simulink model "FW_SkySurfer_HIL"  (R2026b)
settings: Solver=ode4  StopTime=inf  FixedStep=Thil  EnableMultiTasking=on
PreLoadFcn:
  | % Load this folder's HIL settings and MAVLink Bus types (not another project's).
  | run(fullfile(fileparts(get_param(bdroot,'FileName')),'PX4_HIL_preload.m'));
InitFcn:
  | % Record the model first: loading libraries can change the current diagram.
  | assignin('base','lastRunModel',bdroot);
  | % Rebuild HIL settings/Bus types (also after clear all), then aircraft data.
  | hilModelFolder = fileparts(get_param(lastRunModel,'FileName'));
  | run(fullfile(hilModelFolder,'PX4_HIL_preload.m'));
  | run(fullfile(hilModelFolder,'FW_SkySurfer_InitialFunction.m'));
  | clear hilModelFolder
values from neighbouring files (symbols this model uses):
  Aeroelasticity_AIL = [   5   15]    [FW_SkySurfer_InitialFunction.m]
  Aeroelasticity_ELE = [   5   15]    [FW_SkySurfer_InitialFunction.m]
  Aeroelasticity_Gain_AIL = [ 0.8  0.5]    [FW_SkySurfer_InitialFunction.m]
  Aeroelasticity_Gain_ELE = [ 0.9  0.6]    [FW_SkySurfer_InitialFunction.m]
  Aeroelasticity_Gain_RUD = [ 0.9  0.6]    [FW_SkySurfer_InitialFunction.m]
  Aeroelasticity_RUD = [   5   15]    [FW_SkySurfer_InitialFunction.m]
  alpha_avl = [-10 -5 0 5 10 15]    [import_aerostates_avl.m]
  AoA = [-10 -5 0 5 10 15]    [import_aerostates_vsp.m]
  AoS = [-10 0 10]    [import_aerostates_vsp.m]
  b = 1.41    [FW_SkySurfer_InitialFunction.m]
  beta_avl = [-10 -5 0 5 10]    [import_aerostates_avl.m]
  C_wgrp = struct()    [import_aerostates_vsp.m]
  cbar = 0.20    (= 0.2)    [FW_SkySurfer_InitialFunction.m]
  CD_fix_AVL = 0.075    [FW_SkySurfer_InitialFunction.m]
  CD_fix_VSP = 0.065    [FW_SkySurfer_InitialFunction.m]
  CDd01 = zeros(length(mach_avl), length(alpha_avl), length(beta_avl))    [import_aerostates_avl.m]
  CDd02 = zeros(length(mach_avl), length(alpha_avl), length(beta_avl))    [import_aerostates_avl.m]
  CDd03 = zeros(length(mach_avl), length(alpha_avl), length(beta_avl))    [import_aerostates_avl.m]
  CDd04 = zeros(length(mach_avl), length(alpha_avl), length(beta_avl))    [import_aerostates_avl.m]
  CDp = zeros(length(mach_avl), length(alpha_avl), length(beta_avl))    [import_aerostates_avl.m]
  CDq = zeros(length(mach_avl), length(alpha_avl), length(beta_avl))    [import_aerostates_avl.m]
  CDr = zeros(length(mach_avl), length(alpha_avl), length(beta_avl))    [import_aerostates_avl.m]
  CDtot = zeros(length(mach_avl), length(alpha_avl), length(beta_avl))    [import_aerostates_avl.m]
  CG_m = [0.330, 0, 0]    [FW_SkySurfer_InitialFunction.m]
  CLd01 = zeros(length(mach_avl), length(alpha_avl), length(beta_avl))    [import_aerostates_avl.m]
  Cld01 = zeros(length(mach_avl), length(alpha_avl), length(beta_avl))    [import_aerostates_avl.m]
  CLd02 = zeros(length(mach_avl), length(alpha_avl), length(beta_avl))    [import_aerostates_avl.m]
  Cld02 = zeros(length(mach_avl), length(alpha_avl), length(beta_avl))    [import_aerostates_avl.m]
  CLd03 = zeros(length(mach_avl), length(alpha_avl), length(beta_avl))    [import_aerostates_avl.m]
  Cld03 = zeros(length(mach_avl), length(alpha_avl), length(beta_avl))    [import_aerostates_avl.m]
  CLd04 = zeros(length(mach_avl), length(alpha_avl), length(beta_avl))    [import_aerostates_avl.m]
  Cld04 = zeros(length(mach_avl), length(alpha_avl), length(beta_avl))    [import_aerostates_avl.m]
  CLp = zeros(length(mach_avl), length(alpha_avl), length(beta_avl))    [import_aerostates_avl.m]
  Clp = zeros(length(mach_avl), length(alpha_avl), length(beta_avl))    [import_aerostates_avl.m]
  CLq = zeros(length(mach_avl), length(alpha_avl), length(beta_avl))    [import_aerostates_avl.m]
  Clq = zeros(length(mach_avl), length(alpha_avl), length(beta_avl))    [import_aerostates_avl.m]
  CLr = zeros(length(mach_avl), length(alpha_avl), length(beta_avl))    [import_aerostates_avl.m]
  Clr = zeros(length(mach_avl), length(alpha_avl), length(beta_avl))    [import_aerostates_avl.m]
  CLtot = zeros(length(mach_avl), length(alpha_avl), length(beta_avl))    [import_aerostates_avl.m]
  Cltot = zeros(length(mach_avl), length(alpha_avl), length(beta_avl))    [import_aerostates_avl.m]
  Cmd01 = zeros(length(mach_avl), length(alpha_avl), length(beta_avl))    [import_aerostates_avl.m]
  Cmd02 = zeros(length(mach_avl), length(alpha_avl), length(beta_avl))    [import_aerostates_avl.m]
  Cmd03 = zeros(length(mach_avl), length(alpha_avl), length(beta_avl))    [import_aerostates_avl.m]
  Cmd04 = zeros(length(mach_avl), length(alpha_avl), length(beta_avl))    [import_aerostates_avl.m]
  Cmp = zeros(length(mach_avl), length(alpha_avl), length(beta_avl))    [import_aerostates_avl.m]
  Cmq = zeros(length(mach_avl), length(alpha_avl), length(beta_avl))    [import_aerostates_avl.m]
  Cmr = zeros(length(mach_avl), length(alpha_avl), length(beta_avl))    [import_aerostates_avl.m]
  Cmtot = zeros(length(mach_avl), length(alpha_avl), length(beta_avl))    [import_aerostates_avl.m]
  Cnd01 = zeros(length(mach_avl), length(alpha_avl), length(beta_avl))    [import_aerostates_avl.m]
  Cnd02 = zeros(length(mach_avl), length(alpha_avl), length(beta_avl))    [import_aerostates_avl.m]
  Cnd03 = zeros(length(mach_avl), length(alpha_avl), length(beta_avl))    [import_aerostates_avl.m]
  Cnd04 = zeros(length(mach_avl), length(alpha_avl), length(beta_avl))    [import_aerostates_avl.m]
  Cnp = zeros(length(mach_avl), length(alpha_avl), length(beta_avl))    [import_aerostates_avl.m]
  Cnq = zeros(length(mach_avl), length(alpha_avl), length(beta_avl))    [import_aerostates_avl.m]
  Cnr = zeros(length(mach_avl), length(alpha_avl), length(beta_avl))    [import_aerostates_avl.m]
  Cntot = zeros(length(mach_avl), length(alpha_avl), length(beta_avl))    [import_aerostates_avl.m]
  CYd01 = zeros(length(mach_avl), length(alpha_avl), length(beta_avl))    [import_aerostates_avl.m]
  CYd02 = zeros(length(mach_avl), length(alpha_avl), length(beta_avl))    [import_aerostates_avl.m]
  CYd03 = zeros(length(mach_avl), length(alpha_avl), length(beta_avl))    [import_aerostates_avl.m]
  CYd04 = zeros(length(mach_avl), length(alpha_avl), length(beta_avl))    [import_aerostates_avl.m]
  CYp = zeros(length(mach_avl), length(alpha_avl), length(beta_avl))    [import_aerostates_avl.m]
  CYq = zeros(length(mach_avl), length(alpha_avl), length(beta_avl))    [import_aerostates_avl.m]
  CYr = zeros(length(mach_avl), length(alpha_avl), length(beta_avl))    [import_aerostates_avl.m]
  CYtot = zeros(length(mach_avl), length(alpha_avl), length(beta_avl))    [import_aerostates_avl.m]
  del_z = 0    [FW_SkySurfer_InitialFunction.m]
  g = 9.80665    [FW_SkySurfer_InitialFunction.m]
  H0 = 1000 * convlength(1, 'ft', 'm')    [FW_SkySurfer_InitialFunction.m]
  Inertia0 = [  Ixx -Ixy -Ixz  ;                              -Ixy  Iyy -Iyz  ;                              -Ixz -Iyz  Izz ]    [FW_SkySurfer_InitialFunction.m]
  Lat0 = 22.910275834988674    (= 22.910275835)    [FW_SkySurfer_InitialFunction.m]
  Lon0 = 120.31096929726908    (= 120.310969297)    [FW_SkySurfer_InitialFunction.m]
  Mach = [0.05 0.10]    [import_aerostates_vsp.m]
  mach_avl = [0.05 0.10]    [import_aerostates_avl.m]
  Mass0 = 1.3    [FW_SkySurfer_InitialFunction.m]
  Phi0 = 0    [FW_SkySurfer_InitialFunction.m]
  Psi0 = 0    [FW_SkySurfer_InitialFunction.m]
  Psi_w = 0    [FW_SkySurfer_InitialFunction.m]
  Theta0 = 0.8633    [FW_SkySurfer_InitialFunction.m]
  Thil = 1/250    (= 0.004)    [FW_SkySurfer_InitialFunction.m]
  U0 = 40.0309 * convvel(1, 'kts', 'm/s')    [FW_SkySurfer_InitialFunction.m]
  useAVL_VSP = 0    [FW_SkySurfer_InitialFunction.m]
  V0 = 0    [FW_SkySurfer_InitialFunction.m]
  Vel_w = 0    [FW_SkySurfer_InitialFunction.m]
  W0 = 0.6032 * convvel(1, 'kts', 'm/s')    [FW_SkySurfer_InitialFunction.m]
  XREF_m = [0.330, 0, 0]    [FW_SkySurfer_InitialFunction.m]
undefined symbols (not defined in the file or in its folder): F, Light, m, MIL, Newton, Raphson, s, Ts, uavData
libraries: simulink_extras x28, aerolibasang x5, shared6dofsys x4, aerolibwind2 x4, sharedtransform x3, sharedutil x2, shared6dof x2, simulink x1, aerolibatmos2 x1, aerolibconvert2 x1
(part 2 of 3)

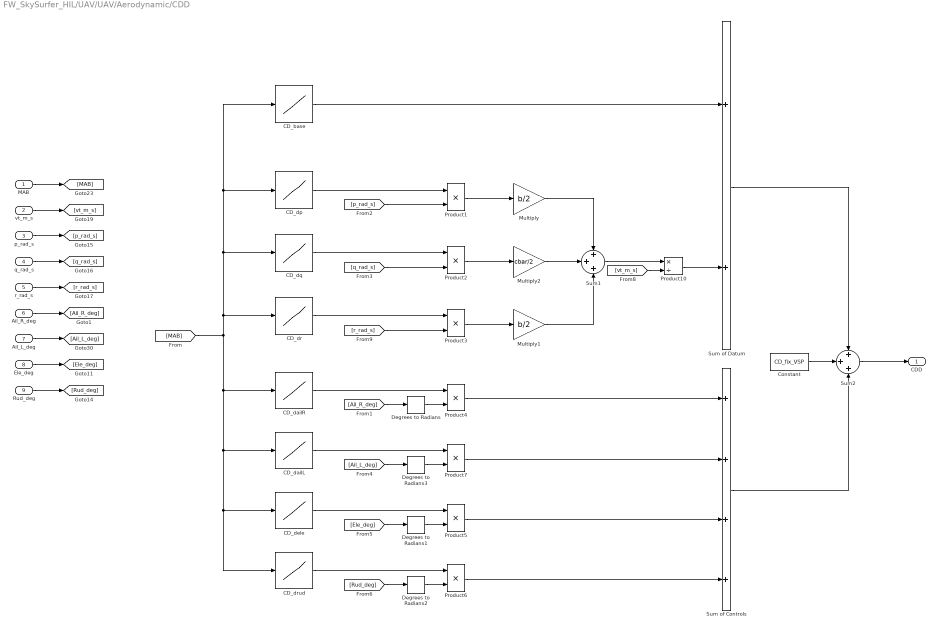
== system FW_SkySurfer_HIL/UAV/UAV/Aerodynamic/CDD ==
  MAB : Inport
  vt_m_s : Inport  Port=2
  p_rad_s : Inport  Port=3
  q_rad_s : Inport  Port=4
  r_rad_s : Inport  Port=5
  Ail_R_deg : Inport  Port=6
  Ail_L_deg : Inport  Port=7
  Ele_deg : Inport  Port=8
  Rud_deg : Inport  Port=9
  CD_base : Lookup_n-D  NumberOfTableDimensions=3  BreakpointsForDimension1=Mach  BreakpointsForDimension2=AoA  BreakpointsForDimension3=AoS  UseOneInputPortForAllInputData=on  Table=C_wgrp.CD_wgrp{1}  InternalRulePriority=Speed  RndMeth=Simplest
  CD_dailL : Lookup_n-D  NumberOfTableDimensions=3  BreakpointsForDimension1=Mach  BreakpointsForDimension2=AoA  BreakpointsForDimension3=AoS  UseOneInputPortForAllInputData=on  Table=C_wgrp.CD_wgrp{10}  InternalRulePriority=Speed  RndMeth=Simplest
  CD_dailR : Lookup_n-D  NumberOfTableDimensions=3  BreakpointsForDimension1=Mach  BreakpointsForDimension2=AoA  BreakpointsForDimension3=AoS  UseOneInputPortForAllInputData=on  Table=C_wgrp.CD_wgrp{9}  InternalRulePriority=Speed  RndMeth=Simplest
  CD_dele : Lookup_n-D  NumberOfTableDimensions=3  BreakpointsForDimension1=Mach  BreakpointsForDimension2=AoA  BreakpointsForDimension3=AoS  UseOneInputPortForAllInputData=on  Table=C_wgrp.CD_wgrp{11}  InternalRulePriority=Speed  RndMeth=Simplest
  CD_dp : Lookup_n-D  NumberOfTableDimensions=3  BreakpointsForDimension1=Mach  BreakpointsForDimension2=AoA  BreakpointsForDimension3=AoS  UseOneInputPortForAllInputData=on  Table=C_wgrp.CD_wgrp{4}  InternalRulePriority=Speed  RndMeth=Simplest
  CD_dq : Lookup_n-D  NumberOfTableDimensions=3  BreakpointsForDimension1=Mach  BreakpointsForDimension2=AoA  BreakpointsForDimension3=AoS  UseOneInputPortForAllInputData=on  Table=C_wgrp.CD_wgrp{5}  InternalRulePriority=Speed  RndMeth=Simplest
  CD_dr : Lookup_n-D  NumberOfTableDimensions=3  BreakpointsForDimension1=Mach  BreakpointsForDimension2=AoA  BreakpointsForDimension3=AoS  UseOneInputPortForAllInputData=on  Table=C_wgrp.CD_wgrp{6}  InternalRulePriority=Speed  RndMeth=Simplest
  CD_drud : Lookup_n-D  NumberOfTableDimensions=3  BreakpointsForDimension1=Mach  BreakpointsForDimension2=AoA  BreakpointsForDimension3=AoS  UseOneInputPortForAllInputData=on  Table=C_wgrp.CD_wgrp{12}  InternalRulePriority=Speed  RndMeth=Simplest
  Constant : Constant  Value=CD_fix_VSP
  Degrees to Radians{,1..3} (4 alike) : simulink_extras/Transformations/Degrees to Radians
  Multiply : Gain  Gain=b/2
  Multiply1 : Gain  Gain=b/2
  Multiply2 : Gain  Gain=cbar/2
  Product{1..7} (7 alike) : Product
  Product10 : Product  Inputs=*/  InputSameDT=on  SaturateOnIntegerOverflow=on  OutDataTypeStr=Inherit: Same as first input
  Sum of Controls : Sum  Inputs=++++
  Sum of Datum : Sum
  Sum1 : Sum  Inputs=+++  InputSameDT=on  SaturateOnIntegerOverflow=on  OutDataTypeStr=Inherit: Same as first input
  Sum2 : Sum  Inputs=+++  InputSameDT=on  SaturateOnIntegerOverflow=on  OutDataTypeStr=Inherit: Same as first input
  CDD : Outport
  wires:
  vt_m_s/1 -> [vt_m_s]
  MAB/1 -> [MAB]
  p_rad_s/1 -> [p_rad_s]
  q_rad_s/1 -> [q_rad_s]
  r_rad_s/1 -> [r_rad_s]
  Ail_R_deg/1 -> [Ail_R_deg]
  Ail_L_deg/1 -> [Ail_L_deg]
  Ele_deg/1 -> [Ele_deg]
  Rud_deg/1 -> [Rud_deg]
  Sum2/1 -> CDD/1
  CD_dailR/1 -> Product4/1
  Multiply/1 -> Sum1/1
  Sum of Controls/1 -> Sum2/3
  Degrees to Radians1/1 -> Product5/2
  Degrees to Radians3/1 -> Product7/2
  CD_drud/1 -> Product6/1
  CD_dr/1 -> Product3/1
  Product7/1 -> Sum of Controls/2
  Product5/1 -> Sum of Controls/3
  CD_dq/1 -> Product2/1
  Sum of Datum/1 -> Sum2/1
  Product3/1 -> Multiply1/1
  CD_dp/1 -> Product1/1
  Multiply2/1 -> Sum1/2
  Degrees to Radians2/1 -> Product6/2
  CD_base/1 -> Sum of Datum/1
  Multiply1/1 -> Sum1/3
  Product6/1 -> Sum of Controls/4
  Product2/1 -> Multiply2/1
  [p_rad_s] -> Product1/2
  Product1/1 -> Multiply/1
  [Ail_L_deg] -> Degrees to Radians3/1
  [Ele_deg] -> Degrees to Radians1/1
  Product10/1 -> Sum of Datum/2
  Degrees to Radians/1 -> Product4/2
  CD_dailL/1 -> Product7/1
  Product4/1 -> Sum of Controls/1
  [Rud_deg] -> Degrees to Radians2/1
  [r_rad_s] -> Product3/2
  [vt_m_s] -> Product10/2
  [MAB] -> CD_dq/1, CD_base/1, CD_dp/1, CD_dr/1, CD_dele/1, CD_drud/1, CD_dailL/1, CD_dailR/1
  CD_dele/1 -> Product5/1
  [q_rad_s] -> Product2/2
  [Ail_R_deg] -> Degrees to Radians/1
  Constant/1 -> Sum2/2
  Sum1/1 -> Product10/1

== system FW_SkySurfer_HIL/UAV/UAV/Aerodynamic/CL ==
  MAB : Inport
  vt_m_s : Inport  Port=2
  p_rad_s : Inport  Port=3
  q_rad_s : Inport  Port=4
  r_rad_s : Inport  Port=5
  Ail_R_deg : Inport  Port=6
  Ail_L_deg : Inport  Port=7
  Ele_deg : Inport  Port=8
  Rud_deg : Inport  Port=9
  CLd01 : Lookup_n-D  NumberOfTableDimensions=3  BreakpointsForDimension1=mach_avl  BreakpointsForDimension2=alpha_avl  BreakpointsForDimension3=beta_avl  UseOneInputPortForAllInputData=on  Table=CLd01  InternalRulePriority=Speed  RndMeth=Simplest
  CLd02 : Lookup_n-D  NumberOfTableDimensions=3  BreakpointsForDimension1=mach_avl  BreakpointsForDimension2=alpha_avl  BreakpointsForDimension3=beta_avl  UseOneInputPortForAllInputData=on  Table=CLd02  InternalRulePriority=Speed  RndMeth=Simplest
  CLd03 : Lookup_n-D  NumberOfTableDimensions=3  BreakpointsForDimension1=mach_avl  BreakpointsForDimension2=alpha_avl  BreakpointsForDimension3=beta_avl  UseOneInputPortForAllInputData=on  Table=CLd03  InternalRulePriority=Speed  RndMeth=Simplest
  CLd04 : Lookup_n-D  NumberOfTableDimensions=3  BreakpointsForDimension1=mach_avl  BreakpointsForDimension2=alpha_avl  BreakpointsForDimension3=beta_avl  UseOneInputPortForAllInputData=on  Table=CLd04  InternalRulePriority=Speed  RndMeth=Simplest
  CLp : Lookup_n-D  NumberOfTableDimensions=3  BreakpointsForDimension1=mach_avl  BreakpointsForDimension2=alpha_avl  BreakpointsForDimension3=beta_avl  UseOneInputPortForAllInputData=on  Table=CLp  InternalRulePriority=Speed  RndMeth=Simplest
  CLq : Lookup_n-D  NumberOfTableDimensions=3  BreakpointsForDimension1=mach_avl  BreakpointsForDimension2=alpha_avl  BreakpointsForDimension3=beta_avl  UseOneInputPortForAllInputData=on  Table=CLq  InternalRulePriority=Speed  RndMeth=Simplest
  CLr : Lookup_n-D  NumberOfTableDimensions=3  BreakpointsForDimension1=mach_avl  BreakpointsForDimension2=alpha_avl  BreakpointsForDimension3=beta_avl  UseOneInputPortForAllInputData=on  Table=CLr  InternalRulePriority=Speed  RndMeth=Simplest
  CLtot : Lookup_n-D  NumberOfTableDimensions=3  BreakpointsForDimension1=mach_avl  BreakpointsForDimension2=alpha_avl  BreakpointsForDimension3=beta_avl  UseOneInputPortForAllInputData=on  Table=CLtot  InternalRulePriority=Speed  RndMeth=Simplest
  Multiply : Gain  Gain=b/2
  Multiply1 : Gain  Gain=b/2
  Multiply2 : Gain  Gain=cbar/2
  Product{1..7} (7 alike) : Product
  Product10 : Product  Inputs=*/  InputSameDT=on  SaturateOnIntegerOverflow=on  OutDataTypeStr=Inherit: Same as first input
  Sum of Controls : Sum  Inputs=++++
  Sum of Datum : Sum
  Sum1 : Sum  Inputs=+++  InputSameDT=on  SaturateOnIntegerOverflow=on  OutDataTypeStr=Inherit: Same as first input
  Sum4 : Sum  InputSameDT=on  SaturateOnIntegerOverflow=on  OutDataTypeStr=Inherit: Same as first input
  CL : Outport
  wires:
  q_rad_s/1 -> [q_rad_s]
  vt_m_s/1 -> [vt_m_s]
  p_rad_s/1 -> [p_rad_s]
  Ail_L_deg/1 -> [Ail_L_deg]
  Ail_R_deg/1 -> [Ail_R_deg]
  MAB/1 -> [MAB]
  r_rad_s/1 -> [r_rad_s]
  Rud_deg/1 -> [Rud_deg]
  Ele_deg/1 -> [Ele_deg]
  [MAB] -> CLr/1, CLq/1, CLp/1, CLtot/1, CLd01/1, CLd02/1, CLd04/1, CLd03/1
  CLd02/1 -> Product7/1
  CLd04/1 -> Product6/1
  Product7/1 -> Sum of Controls/2
  Sum4/1 -> CL/1
  CLd01/1 -> Product4/1
  [r_rad_s] -> Product3/2
  Multiply/1 -> Sum1/1
  Product5/1 -> Sum of Controls/3
  Multiply1/1 -> Sum1/3
  [vt_m_s] -> Product10/2
  Sum of Controls/1 -> Sum4/2
  CLd03/1 -> Product5/1
  Product2/1 -> Multiply2/1
  CLtot/1 -> Sum of Datum/1
  CLq/1 -> Product2/1
  [p_rad_s] -> Product1/2
  Product3/1 -> Multiply1/1
  Product6/1 -> Sum of Controls/4
  Sum of Datum/1 -> Sum4/1
  CLp/1 -> Product1/1
  [q_rad_s] -> Product2/2
  Product1/1 -> Multiply/1
  Multiply2/1 -> Sum1/2
  Product10/1 -> Sum of Datum/2
  CLr/1 -> Product3/1
  Product4/1 -> Sum of Controls/1
  Sum1/1 -> Product10/1
  [Ail_L_deg] -> Product7/2
  [Rud_deg] -> Product6/2
  [Ele_deg] -> Product5/2
  [Ail_R_deg] -> Product4/2

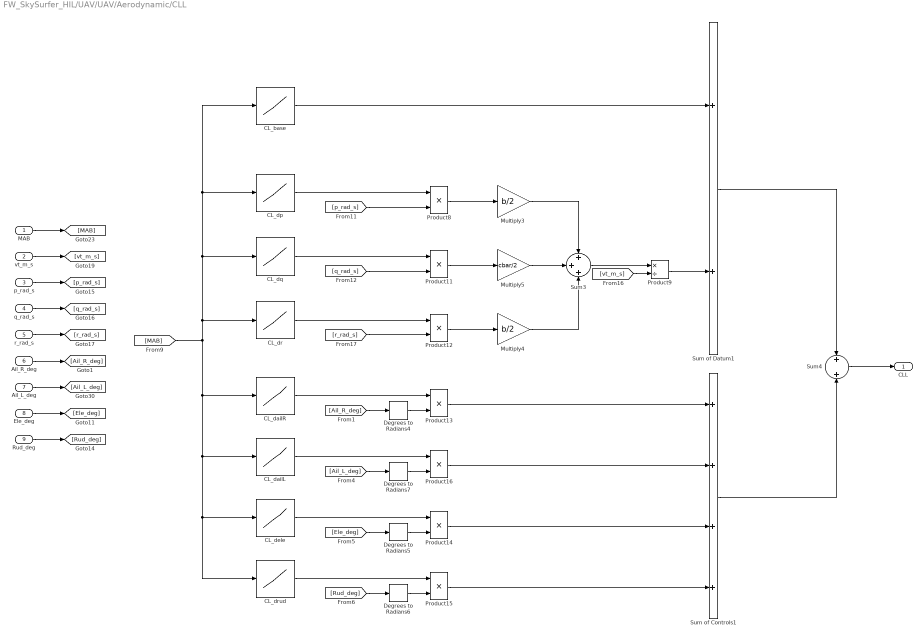
== system FW_SkySurfer_HIL/UAV/UAV/Aerodynamic/CLL ==
  MAB : Inport
  vt_m_s : Inport  Port=2
  p_rad_s : Inport  Port=3
  q_rad_s : Inport  Port=4
  r_rad_s : Inport  Port=5
  Ail_R_deg : Inport  Port=6
  Ail_L_deg : Inport  Port=7
  Ele_deg : Inport  Port=8
  Rud_deg : Inport  Port=9
  CL_base : Lookup_n-D  NumberOfTableDimensions=3  BreakpointsForDimension1=Mach  BreakpointsForDimension2=AoA  BreakpointsForDimension3=AoS  UseOneInputPortForAllInputData=on  Table=C_wgrp.CL_wgrp{1}  InternalRulePriority=Speed  RndMeth=Simplest
  CL_dailL : Lookup_n-D  NumberOfTableDimensions=3  BreakpointsForDimension1=Mach  BreakpointsForDimension2=AoA  BreakpointsForDimension3=AoS  UseOneInputPortForAllInputData=on  Table=C_wgrp.CL_wgrp{10}  InternalRulePriority=Speed  RndMeth=Simplest
  CL_dailR : Lookup_n-D  NumberOfTableDimensions=3  BreakpointsForDimension1=Mach  BreakpointsForDimension2=AoA  BreakpointsForDimension3=AoS  UseOneInputPortForAllInputData=on  Table=C_wgrp.CL_wgrp{9}  InternalRulePriority=Speed  RndMeth=Simplest
  CL_dele : Lookup_n-D  NumberOfTableDimensions=3  BreakpointsForDimension1=Mach  BreakpointsForDimension2=AoA  BreakpointsForDimension3=AoS  UseOneInputPortForAllInputData=on  Table=C_wgrp.CL_wgrp{11}  InternalRulePriority=Speed  RndMeth=Simplest
  CL_dp : Lookup_n-D  NumberOfTableDimensions=3  BreakpointsForDimension1=Mach  BreakpointsForDimension2=AoA  BreakpointsForDimension3=AoS  UseOneInputPortForAllInputData=on  Table=C_wgrp.CL_wgrp{4}  InternalRulePriority=Speed  RndMeth=Simplest
  CL_dq : Lookup_n-D  NumberOfTableDimensions=3  BreakpointsForDimension1=Mach  BreakpointsForDimension2=AoA  BreakpointsForDimension3=AoS  UseOneInputPortForAllInputData=on  Table=C_wgrp.CL_wgrp{5}  InternalRulePriority=Speed  RndMeth=Simplest
  CL_dr : Lookup_n-D  NumberOfTableDimensions=3  BreakpointsForDimension1=Mach  BreakpointsForDimension2=AoA  BreakpointsForDimension3=AoS  UseOneInputPortForAllInputData=on  Table=C_wgrp.CL_wgrp{6}  InternalRulePriority=Speed  RndMeth=Simplest
  CL_drud : Lookup_n-D  NumberOfTableDimensions=3  BreakpointsForDimension1=Mach  BreakpointsForDimension2=AoA  BreakpointsForDimension3=AoS  UseOneInputPortForAllInputData=on  Table=C_wgrp.CL_wgrp{12}  InternalRulePriority=Speed  RndMeth=Simplest
  Degrees to Radians{4..7} (4 alike) : simulink_extras/Transformations/Degrees to Radians
  Multiply3 : Gain  Gain=b/2
  Multiply4 : Gain  Gain=b/2
  Multiply5 : Gain  Gain=cbar/2
  Product{8,11..16} (7 alike) : Product
  Product9 : Product  Inputs=*/  InputSameDT=on  SaturateOnIntegerOverflow=on  OutDataTypeStr=Inherit: Same as first input
  Sum of Controls1 : Sum  Inputs=++++
  Sum of Datum1 : Sum
  Sum3 : Sum  Inputs=+++  InputSameDT=on  SaturateOnIntegerOverflow=on  OutDataTypeStr=Inherit: Same as first input
  Sum4 : Sum  InputSameDT=on  SaturateOnIntegerOverflow=on  OutDataTypeStr=Inherit: Same as first input
  CLL : Outport
  wires:
  Ele_deg/1 -> [Ele_deg]
  q_rad_s/1 -> [q_rad_s]
  p_rad_s/1 -> [p_rad_s]
  r_rad_s/1 -> [r_rad_s]
  MAB/1 -> [MAB]
  vt_m_s/1 -> [vt_m_s]
  Rud_deg/1 -> [Rud_deg]
  Ail_L_deg/1 -> [Ail_L_deg]
  Ail_R_deg/1 -> [Ail_R_deg]
  [r_rad_s] -> Product12/2
  CL_dq/1 -> Product11/1
  Product16/1 -> Sum of Controls1/2
  Sum of Controls1/1 -> Sum4/2
  Degrees to Radians6/1 -> Product15/2
  Product15/1 -> Sum of Controls1/4
  CL_dp/1 -> Product8/1
  Multiply4/1 -> Sum3/3
  Sum of Datum1/1 -> Sum4/1
  CL_dele/1 -> Product14/1
  [Rud_deg] -> Degrees to Radians6/1
  [MAB] -> CL_dr/1, CL_dq/1, CL_dp/1, CL_base/1, CL_dailR/1, CL_dailL/1, CL_drud/1, CL_dele/1
  Product14/1 -> Sum of Controls1/3
  CL_drud/1 -> Product15/1
  CL_base/1 -> Sum of Datum1/1
  [Ele_deg] -> Degrees to Radians5/1
  Product11/1 -> Multiply5/1
  Multiply5/1 -> Sum3/2
  Product9/1 -> Sum of Datum1/2
  [vt_m_s] -> Product9/2
  Degrees to Radians4/1 -> Product13/2
  CL_dailR/1 -> Product13/1
  CL_dr/1 -> Product12/1
  [Ail_R_deg] -> Degrees to Radians4/1
  Product12/1 -> Multiply4/1
  [q_rad_s] -> Product11/2
  Sum3/1 -> Product9/1
  Product8/1 -> Multiply3/1
  Degrees to Radians7/1 -> Product16/2
  Sum4/1 -> CLL/1
  Degrees to Radians5/1 -> Product14/2
  [p_rad_s] -> Product8/2
  [Ail_L_deg] -> Degrees to Radians7/1
  Multiply3/1 -> Sum3/1
  CL_dailL/1 -> Product16/1
  Product13/1 -> Sum of Controls1/1

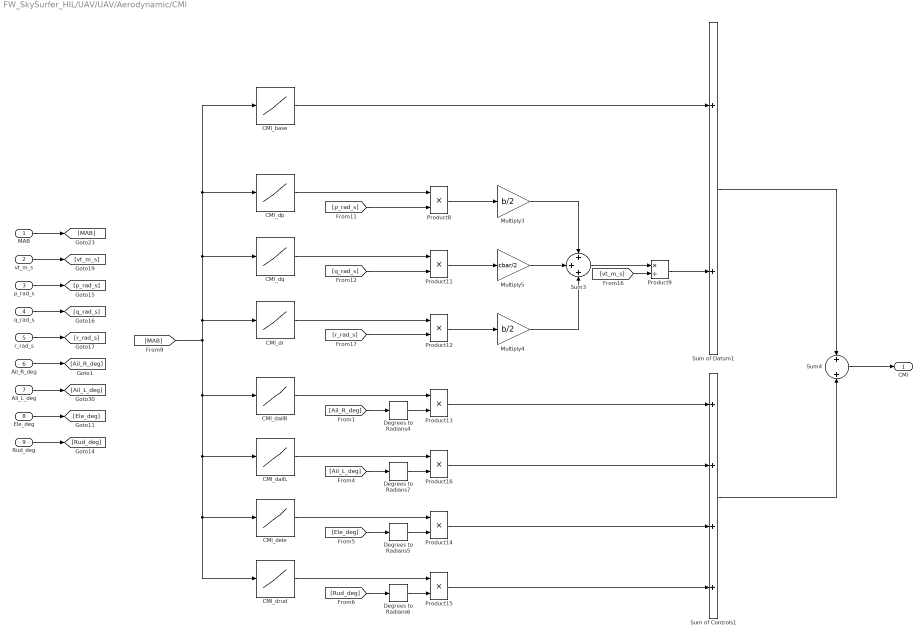
== system FW_SkySurfer_HIL/UAV/UAV/Aerodynamic/CMl ==
  MAB : Inport
  vt_m_s : Inport  Port=2
  p_rad_s : Inport  Port=3
  q_rad_s : Inport  Port=4
  r_rad_s : Inport  Port=5
  Ail_R_deg : Inport  Port=6
  Ail_L_deg : Inport  Port=7
  Ele_deg : Inport  Port=8
  Rud_deg : Inport  Port=9
  CMl_base : Lookup_n-D  NumberOfTableDimensions=3  BreakpointsForDimension1=Mach  BreakpointsForDimension2=AoA  BreakpointsForDimension3=AoS  UseOneInputPortForAllInputData=on  Table=C_wgrp.CMl_wgrp{1}  InternalRulePriority=Speed  RndMeth=Simplest
  CMl_dailL : Lookup_n-D  NumberOfTableDimensions=3  BreakpointsForDimension1=Mach  BreakpointsForDimension2=AoA  BreakpointsForDimension3=AoS  UseOneInputPortForAllInputData=on  Table=C_wgrp.CMl_wgrp{10}  InternalRulePriority=Speed  RndMeth=Simplest
  CMl_dailR : Lookup_n-D  NumberOfTableDimensions=3  BreakpointsForDimension1=Mach  BreakpointsForDimension2=AoA  BreakpointsForDimension3=AoS  UseOneInputPortForAllInputData=on  Table=C_wgrp.CMl_wgrp{9}  InternalRulePriority=Speed  RndMeth=Simplest
  CMl_dele : Lookup_n-D  NumberOfTableDimensions=3  BreakpointsForDimension1=Mach  BreakpointsForDimension2=AoA  BreakpointsForDimension3=AoS  UseOneInputPortForAllInputData=on  Table=C_wgrp.CMl_wgrp{11}  InternalRulePriority=Speed  RndMeth=Simplest
  CMl_dp : Lookup_n-D  NumberOfTableDimensions=3  BreakpointsForDimension1=Mach  BreakpointsForDimension2=AoA  BreakpointsForDimension3=AoS  UseOneInputPortForAllInputData=on  Table=C_wgrp.CMl_wgrp{4}  InternalRulePriority=Speed  RndMeth=Simplest
  CMl_dq : Lookup_n-D  NumberOfTableDimensions=3  BreakpointsForDimension1=Mach  BreakpointsForDimension2=AoA  BreakpointsForDimension3=AoS  UseOneInputPortForAllInputData=on  Table=C_wgrp.CMl_wgrp{5}  InternalRulePriority=Speed  RndMeth=Simplest
  CMl_dr : Lookup_n-D  NumberOfTableDimensions=3  BreakpointsForDimension1=Mach  BreakpointsForDimension2=AoA  BreakpointsForDimension3=AoS  UseOneInputPortForAllInputData=on  Table=C_wgrp.CMl_wgrp{6}  InternalRulePriority=Speed  RndMeth=Simplest
  CMl_drud : Lookup_n-D  NumberOfTableDimensions=3  BreakpointsForDimension1=Mach  BreakpointsForDimension2=AoA  BreakpointsForDimension3=AoS  UseOneInputPortForAllInputData=on  Table=C_wgrp.CMl_wgrp{12}  InternalRulePriority=Speed  RndMeth=Simplest
  Degrees to Radians{4..7} (4 alike) : simulink_extras/Transformations/Degrees to Radians
  Multiply3 : Gain  Gain=b/2
  Multiply4 : Gain  Gain=b/2
  Multiply5 : Gain  Gain=cbar/2
  Product{8,11..16} (7 alike) : Product
  Product9 : Product  Inputs=*/  InputSameDT=on  SaturateOnIntegerOverflow=on  OutDataTypeStr=Inherit: Same as first input
  Sum of Controls1 : Sum  Inputs=++++
  Sum of Datum1 : Sum
  Sum3 : Sum  Inputs=+++  InputSameDT=on  SaturateOnIntegerOverflow=on  OutDataTypeStr=Inherit: Same as first input
  Sum4 : Sum  InputSameDT=on  SaturateOnIntegerOverflow=on  OutDataTypeStr=Inherit: Same as first input
  CMl : Outport
  wires:
  Rud_deg/1 -> [Rud_deg]
  MAB/1 -> [MAB]
  p_rad_s/1 -> [p_rad_s]
  q_rad_s/1 -> [q_rad_s]
  Ail_R_deg/1 -> [Ail_R_deg]
  vt_m_s/1 -> [vt_m_s]
  Ele_deg/1 -> [Ele_deg]
  r_rad_s/1 -> [r_rad_s]
  Ail_L_deg/1 -> [Ail_L_deg]
  Product11/1 -> Multiply5/1
  CMl_dele/1 -> Product14/1
  Degrees to Radians4/1 -> Product13/2
  [Ail_L_deg] -> Degrees to Radians7/1
  Sum of Datum1/1 -> Sum4/1
  CMl_dailL/1 -> Product16/1
  [Rud_deg] -> Degrees to Radians6/1
  Product14/1 -> Sum of Controls1/3
  Sum4/1 -> CMl/1
  [Ail_R_deg] -> Degrees to Radians4/1
  CMl_dq/1 -> Product11/1
  CMl_drud/1 -> Product15/1
  Degrees to Radians6/1 -> Product15/2
  Product8/1 -> Multiply3/1
  [Ele_deg] -> Degrees to Radians5/1
  Multiply3/1 -> Sum3/1
  Degrees to Radians7/1 -> Product16/2
  Sum3/1 -> Product9/1
  [q_rad_s] -> Product11/2
  [r_rad_s] -> Product12/2
  Multiply4/1 -> Sum3/3
  Product9/1 -> Sum of Datum1/2
  [p_rad_s] -> Product8/2
  [MAB] -> CMl_dr/1, CMl_dq/1, CMl_dp/1, CMl_base/1, CMl_drud/1, CMl_dele/1, CMl_dailL/1, CMl_dailR/1
  Product15/1 -> Sum of Controls1/4
  [vt_m_s] -> Product9/2
  CMl_dp/1 -> Product8/1
  CMl_base/1 -> Sum of Datum1/1
  CMl_dr/1 -> Product12/1
  Degrees to Radians5/1 -> Product14/2
  Product12/1 -> Multiply4/1
  Multiply5/1 -> Sum3/2
  CMl_dailR/1 -> Product13/1
  Sum of Controls1/1 -> Sum4/2
  Product13/1 -> Sum of Controls1/1
  Product16/1 -> Sum of Controls1/2

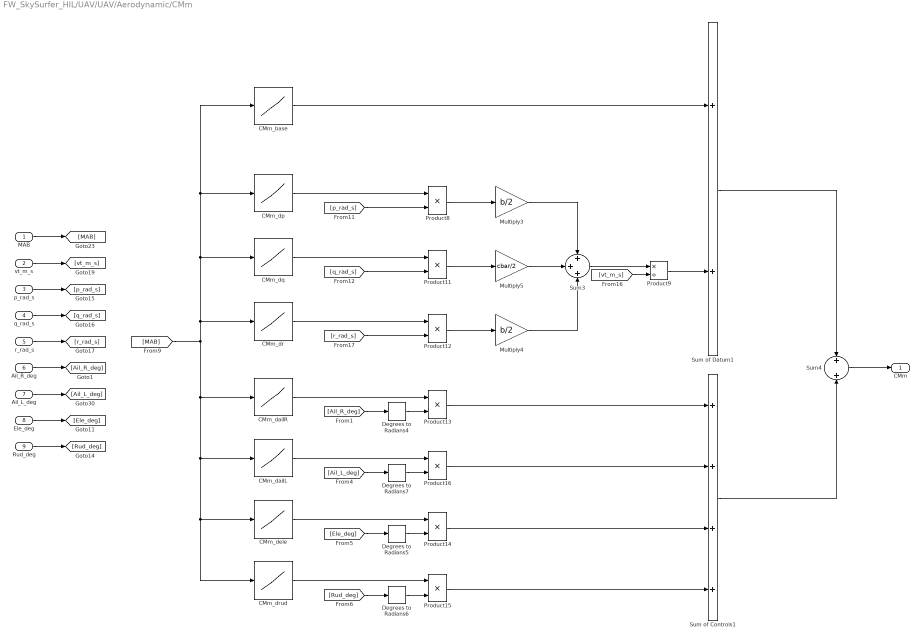
== system FW_SkySurfer_HIL/UAV/UAV/Aerodynamic/CMm ==
  MAB : Inport
  vt_m_s : Inport  Port=2
  p_rad_s : Inport  Port=3
  q_rad_s : Inport  Port=4
  r_rad_s : Inport  Port=5
  Ail_R_deg : Inport  Port=6
  Ail_L_deg : Inport  Port=7
  Ele_deg : Inport  Port=8
  Rud_deg : Inport  Port=9
  CMm_base : Lookup_n-D  NumberOfTableDimensions=3  BreakpointsForDimension1=Mach  BreakpointsForDimension2=AoA  BreakpointsForDimension3=AoS  UseOneInputPortForAllInputData=on  Table=C_wgrp.CMm_wgrp{1}  InternalRulePriority=Speed  RndMeth=Simplest
  CMm_dailL : Lookup_n-D  NumberOfTableDimensions=3  BreakpointsForDimension1=Mach  BreakpointsForDimension2=AoA  BreakpointsForDimension3=AoS  UseOneInputPortForAllInputData=on  Table=C_wgrp.CMm_wgrp{10}  InternalRulePriority=Speed  RndMeth=Simplest
  CMm_dailR : Lookup_n-D  NumberOfTableDimensions=3  BreakpointsForDimension1=Mach  BreakpointsForDimension2=AoA  BreakpointsForDimension3=AoS  UseOneInputPortForAllInputData=on  Table=C_wgrp.CMm_wgrp{9}  InternalRulePriority=Speed  RndMeth=Simplest
  CMm_dele : Lookup_n-D  NumberOfTableDimensions=3  BreakpointsForDimension1=Mach  BreakpointsForDimension2=AoA  BreakpointsForDimension3=AoS  UseOneInputPortForAllInputData=on  Table=C_wgrp.CMm_wgrp{11}  InternalRulePriority=Speed  RndMeth=Simplest
  CMm_dp : Lookup_n-D  NumberOfTableDimensions=3  BreakpointsForDimension1=Mach  BreakpointsForDimension2=AoA  BreakpointsForDimension3=AoS  UseOneInputPortForAllInputData=on  Table=C_wgrp.CMm_wgrp{4}  InternalRulePriority=Speed  RndMeth=Simplest
  CMm_dq : Lookup_n-D  NumberOfTableDimensions=3  BreakpointsForDimension1=Mach  BreakpointsForDimension2=AoA  BreakpointsForDimension3=AoS  UseOneInputPortForAllInputData=on  Table=C_wgrp.CMm_wgrp{5}  InternalRulePriority=Speed  RndMeth=Simplest
  CMm_dr : Lookup_n-D  NumberOfTableDimensions=3  BreakpointsForDimension1=Mach  BreakpointsForDimension2=AoA  BreakpointsForDimension3=AoS  UseOneInputPortForAllInputData=on  Table=C_wgrp.CMm_wgrp{6}  InternalRulePriority=Speed  RndMeth=Simplest
  CMm_drud : Lookup_n-D  NumberOfTableDimensions=3  BreakpointsForDimension1=Mach  BreakpointsForDimension2=AoA  BreakpointsForDimension3=AoS  UseOneInputPortForAllInputData=on  Table=C_wgrp.CMm_wgrp{12}  InternalRulePriority=Speed  RndMeth=Simplest
  Degrees to Radians{4..7} (4 alike) : simulink_extras/Transformations/Degrees to Radians
  Multiply3 : Gain  Gain=b/2
  Multiply4 : Gain  Gain=b/2
  Multiply5 : Gain  Gain=cbar/2
  Product{8,11..16} (7 alike) : Product
  Product9 : Product  Inputs=*/  InputSameDT=on  SaturateOnIntegerOverflow=on  OutDataTypeStr=Inherit: Same as first input
  Sum of Controls1 : Sum  Inputs=++++
  Sum of Datum1 : Sum
  Sum3 : Sum  Inputs=+++  InputSameDT=on  SaturateOnIntegerOverflow=on  OutDataTypeStr=Inherit: Same as first input
  Sum4 : Sum  InputSameDT=on  SaturateOnIntegerOverflow=on  OutDataTypeStr=Inherit: Same as first input
  CMm : Outport
  wires:
  Rud_deg/1 -> [Rud_deg]
  MAB/1 -> [MAB]
  p_rad_s/1 -> [p_rad_s]
  q_rad_s/1 -> [q_rad_s]
  Ail_R_deg/1 -> [Ail_R_deg]
  vt_m_s/1 -> [vt_m_s]
  Ele_deg/1 -> [Ele_deg]
  r_rad_s/1 -> [r_rad_s]
  Ail_L_deg/1 -> [Ail_L_deg]
  [r_rad_s] -> Product12/2
  CMm_dele/1 -> Product14/1
  Product11/1 -> Multiply5/1
  CMm_base/1 -> Sum of Datum1/1
  Product13/1 -> Sum of Controls1/1
  [Ail_R_deg] -> Degrees to Radians4/1
  CMm_dq/1 -> Product11/1
  Multiply4/1 -> Sum3/3
  Product16/1 -> Sum of Controls1/2
  Sum of Controls1/1 -> Sum4/2
  CMm_dailR/1 -> Product13/1
  Degrees to Radians6/1 -> Product15/2
  Sum of Datum1/1 -> Sum4/1
  [vt_m_s] -> Product9/2
  Sum4/1 -> CMm/1
  Degrees to Radians7/1 -> Product16/2
  [Ail_L_deg] -> Degrees to Radians7/1
  Product9/1 -> Sum of Datum1/2
  Sum3/1 -> Product9/1
  [q_rad_s] -> Product11/2
  Product8/1 -> Multiply3/1
  CMm_dp/1 -> Product8/1
  CMm_drud/1 -> Product15/1
  [Ele_deg] -> Degrees to Radians5/1
  Product12/1 -> Multiply4/1
  Product15/1 -> Sum of Controls1/4
  [MAB] -> CMm_dr/1, CMm_dq/1, CMm_dp/1, CMm_base/1, CMm_dailR/1, CMm_dailL/1, CMm_drud/1, CMm_dele/1
  [Rud_deg] -> Degrees to Radians6/1
  [p_rad_s] -> Product8/2
  Multiply3/1 -> Sum3/1
  Multiply5/1 -> Sum3/2
  CMm_dailL/1 -> Product16/1
  Degrees to Radians5/1 -> Product14/2
  CMm_dr/1 -> Product12/1
  Product14/1 -> Sum of Controls1/3
  Degrees to Radians4/1 -> Product13/2

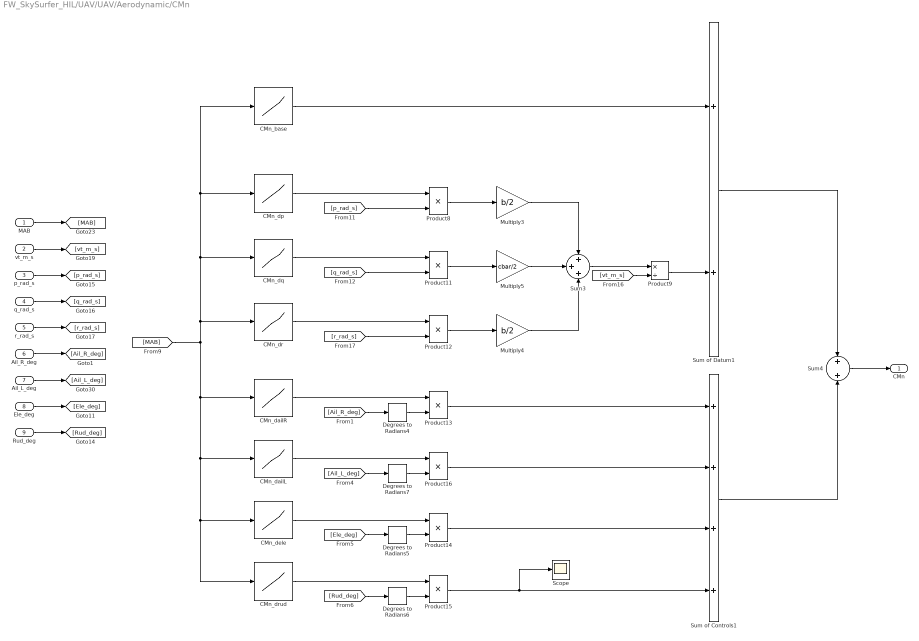
== system FW_SkySurfer_HIL/UAV/UAV/Aerodynamic/CMn ==
  MAB : Inport
  vt_m_s : Inport  Port=2
  p_rad_s : Inport  Port=3
  q_rad_s : Inport  Port=4
  r_rad_s : Inport  Port=5
  Ail_R_deg : Inport  Port=6
  Ail_L_deg : Inport  Port=7
  Ele_deg : Inport  Port=8
  Rud_deg : Inport  Port=9
  CMn_base : Lookup_n-D  NumberOfTableDimensions=3  BreakpointsForDimension1=Mach  BreakpointsForDimension2=AoA  BreakpointsForDimension3=AoS  UseOneInputPortForAllInputData=on  Table=C_wgrp.CMn_wgrp{1}  InternalRulePriority=Speed  RndMeth=Simplest
  CMn_dailL : Lookup_n-D  NumberOfTableDimensions=3  BreakpointsForDimension1=Mach  BreakpointsForDimension2=AoA  BreakpointsForDimension3=AoS  UseOneInputPortForAllInputData=on  Table=C_wgrp.CMn_wgrp{10}  InternalRulePriority=Speed  RndMeth=Simplest
  CMn_dailR : Lookup_n-D  NumberOfTableDimensions=3  BreakpointsForDimension1=Mach  BreakpointsForDimension2=AoA  BreakpointsForDimension3=AoS  UseOneInputPortForAllInputData=on  Table=C_wgrp.CMn_wgrp{9}  InternalRulePriority=Speed  RndMeth=Simplest
  CMn_dele : Lookup_n-D  NumberOfTableDimensions=3  BreakpointsForDimension1=Mach  BreakpointsForDimension2=AoA  BreakpointsForDimension3=AoS  UseOneInputPortForAllInputData=on  Table=C_wgrp.CMn_wgrp{11}  InternalRulePriority=Speed  RndMeth=Simplest
  CMn_dp : Lookup_n-D  NumberOfTableDimensions=3  BreakpointsForDimension1=Mach  BreakpointsForDimension2=AoA  BreakpointsForDimension3=AoS  UseOneInputPortForAllInputData=on  Table=C_wgrp.CMn_wgrp{4}  InternalRulePriority=Speed  RndMeth=Simplest
  CMn_dq : Lookup_n-D  NumberOfTableDimensions=3  BreakpointsForDimension1=Mach  BreakpointsForDimension2=AoA  BreakpointsForDimension3=AoS  UseOneInputPortForAllInputData=on  Table=C_wgrp.CMn_wgrp{5}  InternalRulePriority=Speed  RndMeth=Simplest
  CMn_dr : Lookup_n-D  NumberOfTableDimensions=3  BreakpointsForDimension1=Mach  BreakpointsForDimension2=AoA  BreakpointsForDimension3=AoS  UseOneInputPortForAllInputData=on  Table=C_wgrp.CMn_wgrp{6}  InternalRulePriority=Speed  RndMeth=Simplest
  CMn_drud : Lookup_n-D  NumberOfTableDimensions=3  BreakpointsForDimension1=Mach  BreakpointsForDimension2=AoA  BreakpointsForDimension3=AoS  UseOneInputPortForAllInputData=on  Table=C_wgrp.CMn_wgrp{12}  InternalRulePriority=Speed  RndMeth=Simplest
  Degrees to Radians{4..7} (4 alike) : simulink_extras/Transformations/Degrees to Radians
  Multiply3 : Gain  Gain=b/2
  Multiply4 : Gain  Gain=b/2
  Multiply5 : Gain  Gain=cbar/2
  Product{8,11..16} (7 alike) : Product
  Product9 : Product  Inputs=*/  InputSameDT=on  SaturateOnIntegerOverflow=on  OutDataTypeStr=Inherit: Same as first input
  Scope : Scope
      settings: ActiveDisplayYMinimum=-1  ActiveDisplayYMaximum=1  DataLoggingVariableName=ScopeData24
  Sum of Controls1 : Sum  Inputs=++++
  Sum of Datum1 : Sum
  Sum3 : Sum  Inputs=+++  InputSameDT=on  SaturateOnIntegerOverflow=on  OutDataTypeStr=Inherit: Same as first input
  Sum4 : Sum  InputSameDT=on  SaturateOnIntegerOverflow=on  OutDataTypeStr=Inherit: Same as first input
  CMn : Outport
  wires:
  Rud_deg/1 -> [Rud_deg]
  MAB/1 -> [MAB]
  p_rad_s/1 -> [p_rad_s]
  q_rad_s/1 -> [q_rad_s]
  Ail_R_deg/1 -> [Ail_R_deg]
  vt_m_s/1 -> [vt_m_s]
  Ele_deg/1 -> [Ele_deg]
  r_rad_s/1 -> [r_rad_s]
  Ail_L_deg/1 -> [Ail_L_deg]
  CMn_dq/1 -> Product11/1
  CMn_dp/1 -> Product8/1
  Product8/1 -> Multiply3/1
  Multiply3/1 -> Sum3/1
  [p_rad_s] -> Product8/2
  Sum3/1 -> Product9/1
  [Ele_deg] -> Degrees to Radians5/1
  Sum of Controls1/1 -> Sum4/2
  Multiply4/1 -> Sum3/3
  Product15/1 -> Scope/1, Sum of Controls1/4
  Sum4/1 -> CMn/1
  Product12/1 -> Multiply4/1
  Product16/1 -> Sum of Controls1/2
  [r_rad_s] -> Product12/2
  Degrees to Radians7/1 -> Product16/2
  Multiply5/1 -> Sum3/2
  CMn_dele/1 -> Product14/1
  Sum of Datum1/1 -> Sum4/1
  [vt_m_s] -> Product9/2
  Degrees to Radians5/1 -> Product14/2
  CMn_dailR/1 -> Product13/1
  Degrees to Radians6/1 -> Product15/2
  [Rud_deg] -> Degrees to Radians6/1
  CMn_dr/1 -> Product12/1
  CMn_base/1 -> Sum of Datum1/1
  Degrees to Radians4/1 -> Product13/2
  [Ail_L_deg] -> Degrees to Radians7/1
  CMn_dailL/1 -> Product16/1
  Product14/1 -> Sum of Controls1/3
  Product13/1 -> Sum of Controls1/1
  CMn_drud/1 -> Product15/1
  Product9/1 -> Sum of Datum1/2
  [MAB] -> CMn_dr/1, CMn_dq/1, CMn_dp/1, CMn_base/1, CMn_dailR/1, CMn_dailL/1, CMn_drud/1, CMn_dele/1
  [Ail_R_deg] -> Degrees to Radians4/1
  Product11/1 -> Multiply5/1
  [q_rad_s] -> Product11/2

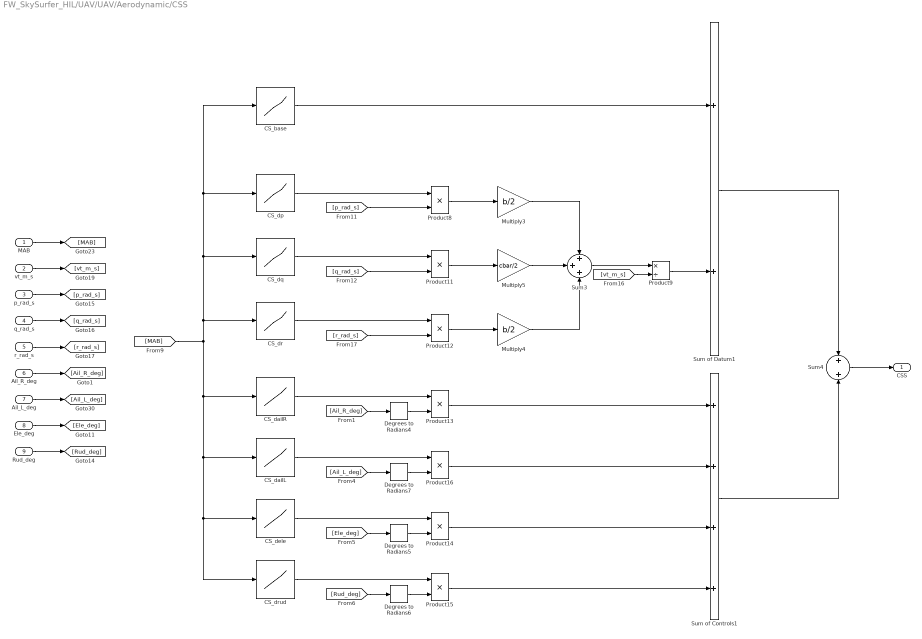
== system FW_SkySurfer_HIL/UAV/UAV/Aerodynamic/CSS ==
  MAB : Inport
  vt_m_s : Inport  Port=2
  p_rad_s : Inport  Port=3
  q_rad_s : Inport  Port=4
  r_rad_s : Inport  Port=5
  Ail_R_deg : Inport  Port=6
  Ail_L_deg : Inport  Port=7
  Ele_deg : Inport  Port=8
  Rud_deg : Inport  Port=9
  CS_base : Lookup_n-D  NumberOfTableDimensions=3  BreakpointsForDimension1=Mach  BreakpointsForDimension2=AoA  BreakpointsForDimension3=AoS  UseOneInputPortForAllInputData=on  Table=C_wgrp.CS_wgrp{1}  InternalRulePriority=Speed  RndMeth=Simplest
  CS_dailL : Lookup_n-D  NumberOfTableDimensions=3  BreakpointsForDimension1=Mach  BreakpointsForDimension2=AoA  BreakpointsForDimension3=AoS  UseOneInputPortForAllInputData=on  Table=C_wgrp.CS_wgrp{10}  InternalRulePriority=Speed  RndMeth=Simplest
  CS_dailR : Lookup_n-D  NumberOfTableDimensions=3  BreakpointsForDimension1=Mach  BreakpointsForDimension2=AoA  BreakpointsForDimension3=AoS  UseOneInputPortForAllInputData=on  Table=C_wgrp.CS_wgrp{9}  InternalRulePriority=Speed  RndMeth=Simplest
  CS_dele : Lookup_n-D  NumberOfTableDimensions=3  BreakpointsForDimension1=Mach  BreakpointsForDimension2=AoA  BreakpointsForDimension3=AoS  UseOneInputPortForAllInputData=on  Table=C_wgrp.CS_wgrp{11}  InternalRulePriority=Speed  RndMeth=Simplest
  CS_dp : Lookup_n-D  NumberOfTableDimensions=3  BreakpointsForDimension1=Mach  BreakpointsForDimension2=AoA  BreakpointsForDimension3=AoS  UseOneInputPortForAllInputData=on  Table=C_wgrp.CS_wgrp{4}  InternalRulePriority=Speed  RndMeth=Simplest
  CS_dq : Lookup_n-D  NumberOfTableDimensions=3  BreakpointsForDimension1=Mach  BreakpointsForDimension2=AoA  BreakpointsForDimension3=AoS  UseOneInputPortForAllInputData=on  Table=C_wgrp.CS_wgrp{5}  InternalRulePriority=Speed  RndMeth=Simplest
  CS_dr : Lookup_n-D  NumberOfTableDimensions=3  BreakpointsForDimension1=Mach  BreakpointsForDimension2=AoA  BreakpointsForDimension3=AoS  UseOneInputPortForAllInputData=on  Table=C_wgrp.CS_wgrp{6}  InternalRulePriority=Speed  RndMeth=Simplest
  CS_drud : Lookup_n-D  NumberOfTableDimensions=3  BreakpointsForDimension1=Mach  BreakpointsForDimension2=AoA  BreakpointsForDimension3=AoS  UseOneInputPortForAllInputData=on  Table=C_wgrp.CS_wgrp{12}  InternalRulePriority=Speed  RndMeth=Simplest
  Degrees to Radians{4..7} (4 alike) : simulink_extras/Transformations/Degrees to Radians
  Multiply3 : Gain  Gain=b/2
  Multiply4 : Gain  Gain=b/2
  Multiply5 : Gain  Gain=cbar/2
  Product{8,11..16} (7 alike) : Product
  Product9 : Product  Inputs=*/  InputSameDT=on  SaturateOnIntegerOverflow=on  OutDataTypeStr=Inherit: Same as first input
  Sum of Controls1 : Sum  Inputs=++++
  Sum of Datum1 : Sum
  Sum3 : Sum  Inputs=+++  InputSameDT=on  SaturateOnIntegerOverflow=on  OutDataTypeStr=Inherit: Same as first input
  Sum4 : Sum  InputSameDT=on  SaturateOnIntegerOverflow=on  OutDataTypeStr=Inherit: Same as first input
  CSS : Outport
  wires:
  Ele_deg/1 -> [Ele_deg]
  q_rad_s/1 -> [q_rad_s]
  p_rad_s/1 -> [p_rad_s]
  r_rad_s/1 -> [r_rad_s]
  MAB/1 -> [MAB]
  vt_m_s/1 -> [vt_m_s]
  Rud_deg/1 -> [Rud_deg]
  Ail_L_deg/1 -> [Ail_L_deg]
  Ail_R_deg/1 -> [Ail_R_deg]
  [p_rad_s] -> Product8/2
  CS_dq/1 -> Product11/1
  [Rud_deg] -> Degrees to Radians6/1
  Product8/1 -> Multiply3/1
  CS_dr/1 -> Product12/1
  Sum of Datum1/1 -> Sum4/1
  Degrees to Radians7/1 -> Product16/2
  [Ail_L_deg] -> Degrees to Radians7/1
  [Ail_R_deg] -> Degrees to Radians4/1
  Sum3/1 -> Product9/1
  [MAB] -> CS_dr/1, CS_dq/1, CS_dp/1, CS_base/1, CS_dailR/1, CS_dailL/1, CS_drud/1, CS_dele/1
  Sum4/1 -> CSS/1
  CS_drud/1 -> Product15/1
  Product11/1 -> Multiply5/1
  [Ele_deg] -> Degrees to Radians5/1
  CS_dailL/1 -> Product16/1
  Degrees to Radians5/1 -> Product14/2
  Multiply4/1 -> Sum3/3
  CS_dailR/1 -> Product13/1
  Multiply3/1 -> Sum3/1
  Product16/1 -> Sum of Controls1/2
  CS_base/1 -> Sum of Datum1/1
  Degrees to Radians4/1 -> Product13/2
  [vt_m_s] -> Product9/2
  Product12/1 -> Multiply4/1
  CS_dp/1 -> Product8/1
  Product9/1 -> Sum of Datum1/2
  Sum of Controls1/1 -> Sum4/2
  CS_dele/1 -> Product14/1
  Product13/1 -> Sum of Controls1/1
  Product14/1 -> Sum of Controls1/3
  Multiply5/1 -> Sum3/2
  [q_rad_s] -> Product11/2
  [r_rad_s] -> Product12/2
  Degrees to Radians6/1 -> Product15/2
  Product15/1 -> Sum of Controls1/4

== system FW_SkySurfer_HIL/UAV/UAV/Aerodynamic/CY ==
  MAB : Inport
  vt_m_s : Inport  Port=2
  p_rad_s : Inport  Port=3
  q_rad_s : Inport  Port=4
  r_rad_s : Inport  Port=5
  Ail_R_deg : Inport  Port=6
  Ail_L_deg : Inport  Port=7
  Ele_deg : Inport  Port=8
  Rud_deg : Inport  Port=9
  CYd01 : Lookup_n-D  NumberOfTableDimensions=3  BreakpointsForDimension1=mach_avl  BreakpointsForDimension2=alpha_avl  BreakpointsForDimension3=beta_avl  UseOneInputPortForAllInputData=on  Table=CYd01  InternalRulePriority=Speed  RndMeth=Simplest
  CYd02 : Lookup_n-D  NumberOfTableDimensions=3  BreakpointsForDimension1=mach_avl  BreakpointsForDimension2=alpha_avl  BreakpointsForDimension3=beta_avl  UseOneInputPortForAllInputData=on  Table=CYd02  InternalRulePriority=Speed  RndMeth=Simplest
  CYd03 : Lookup_n-D  NumberOfTableDimensions=3  BreakpointsForDimension1=mach_avl  BreakpointsForDimension2=alpha_avl  BreakpointsForDimension3=beta_avl  UseOneInputPortForAllInputData=on  Table=CYd03  InternalRulePriority=Speed  RndMeth=Simplest
  CYd04 : Lookup_n-D  NumberOfTableDimensions=3  BreakpointsForDimension1=mach_avl  BreakpointsForDimension2=alpha_avl  BreakpointsForDimension3=beta_avl  UseOneInputPortForAllInputData=on  Table=CYd04  InternalRulePriority=Speed  RndMeth=Simplest
  CYp : Lookup_n-D  NumberOfTableDimensions=3  BreakpointsForDimension1=mach_avl  BreakpointsForDimension2=alpha_avl  BreakpointsForDimension3=beta_avl  UseOneInputPortForAllInputData=on  Table=CYp  InternalRulePriority=Speed  RndMeth=Simplest
  CYq : Lookup_n-D  NumberOfTableDimensions=3  BreakpointsForDimension1=mach_avl  BreakpointsForDimension2=alpha_avl  BreakpointsForDimension3=beta_avl  UseOneInputPortForAllInputData=on  Table=CYq  InternalRulePriority=Speed  RndMeth=Simplest
  CYr : Lookup_n-D  NumberOfTableDimensions=3  BreakpointsForDimension1=mach_avl  BreakpointsForDimension2=alpha_avl  BreakpointsForDimension3=beta_avl  UseOneInputPortForAllInputData=on  Table=CYr  InternalRulePriority=Speed  RndMeth=Simplest
  CYtot : Lookup_n-D  NumberOfTableDimensions=3  BreakpointsForDimension1=mach_avl  BreakpointsForDimension2=alpha_avl  BreakpointsForDimension3=beta_avl  UseOneInputPortForAllInputData=on  Table=CYtot  InternalRulePriority=Speed  RndMeth=Simplest
  Multiply : Gain  Gain=b/2
  Multiply1 : Gain  Gain=b/2
  Multiply2 : Gain  Gain=cbar/2
  Product{1..7} (7 alike) : Product
  Product10 : Product  Inputs=*/  InputSameDT=on  SaturateOnIntegerOverflow=on  OutDataTypeStr=Inherit: Same as first input
  Sum of Controls : Sum  Inputs=++++
  Sum of Datum : Sum
  Sum1 : Sum  Inputs=+++  InputSameDT=on  SaturateOnIntegerOverflow=on  OutDataTypeStr=Inherit: Same as first input
  Sum4 : Sum  InputSameDT=on  SaturateOnIntegerOverflow=on  OutDataTypeStr=Inherit: Same as first input
  CY : Outport
  wires:
  q_rad_s/1 -> [q_rad_s]
  vt_m_s/1 -> [vt_m_s]
  p_rad_s/1 -> [p_rad_s]
  Ail_L_deg/1 -> [Ail_L_deg]
  Ail_R_deg/1 -> [Ail_R_deg]
  MAB/1 -> [MAB]
  r_rad_s/1 -> [r_rad_s]
  Rud_deg/1 -> [Rud_deg]
  Ele_deg/1 -> [Ele_deg]
  CYd02/1 -> Product7/1
  Product10/1 -> Sum of Datum/2
  Product3/1 -> Multiply1/1
  CYd04/1 -> Product6/1
  CYr/1 -> Product3/1
  CYq/1 -> Product2/1
  Product6/1 -> Sum of Controls/4
  Multiply2/1 -> Sum1/2
  Sum of Datum/1 -> Sum4/1
  Sum of Controls/1 -> Sum4/2
  CYp/1 -> Product1/1
  CYd03/1 -> Product5/1
  Product4/1 -> Sum of Controls/1
  Sum1/1 -> Product10/1
  Sum4/1 -> CY/1
  CYtot/1 -> Sum of Datum/1
  Product2/1 -> Multiply2/1
  CYd01/1 -> Product4/1
  [p_rad_s] -> Product1/2
  [q_rad_s] -> Product2/2
  [r_rad_s] -> Product3/2
  [vt_m_s] -> Product10/2
  Product1/1 -> Multiply/1
  Product7/1 -> Sum of Controls/2
  [MAB] -> CYr/1, CYq/1, CYp/1, CYtot/1, CYd01/1, CYd02/1, CYd04/1, CYd03/1
  Product5/1 -> Sum of Controls/3
  Multiply1/1 -> Sum1/3
  Multiply/1 -> Sum1/1
  [Ail_L_deg] -> Product7/2
  [Rud_deg] -> Product6/2
  [Ele_deg] -> Product5/2
  [Ail_R_deg] -> Product4/2

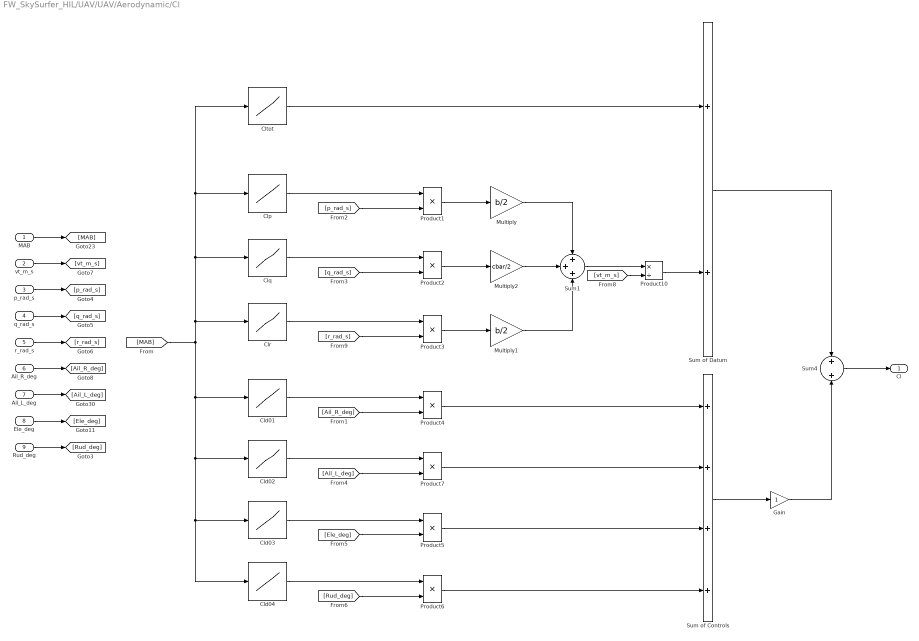
== system FW_SkySurfer_HIL/UAV/UAV/Aerodynamic/Cl ==
  MAB : Inport
  vt_m_s : Inport  Port=2
  p_rad_s : Inport  Port=3
  q_rad_s : Inport  Port=4
  r_rad_s : Inport  Port=5
  Ail_R_deg : Inport  Port=6
  Ail_L_deg : Inport  Port=7
  Ele_deg : Inport  Port=8
  Rud_deg : Inport  Port=9
  Cld01 : Lookup_n-D  NumberOfTableDimensions=3  BreakpointsForDimension1=mach_avl  BreakpointsForDimension2=alpha_avl  BreakpointsForDimension3=beta_avl  UseOneInputPortForAllInputData=on  Table=Cld01  InternalRulePriority=Speed  RndMeth=Simplest
  Cld02 : Lookup_n-D  NumberOfTableDimensions=3  BreakpointsForDimension1=mach_avl  BreakpointsForDimension2=alpha_avl  BreakpointsForDimension3=beta_avl  UseOneInputPortForAllInputData=on  Table=Cld02  InternalRulePriority=Speed  RndMeth=Simplest
  Cld03 : Lookup_n-D  NumberOfTableDimensions=3  BreakpointsForDimension1=mach_avl  BreakpointsForDimension2=alpha_avl  BreakpointsForDimension3=beta_avl  UseOneInputPortForAllInputData=on  Table=Cld03  InternalRulePriority=Speed  RndMeth=Simplest
  Cld04 : Lookup_n-D  NumberOfTableDimensions=3  BreakpointsForDimension1=mach_avl  BreakpointsForDimension2=alpha_avl  BreakpointsForDimension3=beta_avl  UseOneInputPortForAllInputData=on  Table=Cld04  InternalRulePriority=Speed  RndMeth=Simplest
  Clp : Lookup_n-D  NumberOfTableDimensions=3  BreakpointsForDimension1=mach_avl  BreakpointsForDimension2=alpha_avl  BreakpointsForDimension3=beta_avl  UseOneInputPortForAllInputData=on  Table=Clp  InternalRulePriority=Speed  RndMeth=Simplest
  Clq : Lookup_n-D  NumberOfTableDimensions=3  BreakpointsForDimension1=mach_avl  BreakpointsForDimension2=alpha_avl  BreakpointsForDimension3=beta_avl  UseOneInputPortForAllInputData=on  Table=Clq  InternalRulePriority=Speed  RndMeth=Simplest
  Clr : Lookup_n-D  NumberOfTableDimensions=3  BreakpointsForDimension1=mach_avl  BreakpointsForDimension2=alpha_avl  BreakpointsForDimension3=beta_avl  UseOneInputPortForAllInputData=on  Table=Clr  InternalRulePriority=Speed  RndMeth=Simplest
  Cltot : Lookup_n-D  NumberOfTableDimensions=3  BreakpointsForDimension1=mach_avl  BreakpointsForDimension2=alpha_avl  BreakpointsForDimension3=beta_avl  UseOneInputPortForAllInputData=on  Table=Cltot  InternalRulePriority=Speed  RndMeth=Simplest
  Gain : Gain
  Multiply : Gain  Gain=b/2
  Multiply1 : Gain  Gain=b/2
  Multiply2 : Gain  Gain=cbar/2
  Product{1..7} (7 alike) : Product
  Product10 : Product  Inputs=*/  InputSameDT=on  SaturateOnIntegerOverflow=on  OutDataTypeStr=Inherit: Same as first input
  Sum of Controls : Sum  Inputs=++++
  Sum of Datum : Sum
  Sum1 : Sum  Inputs=+++  InputSameDT=on  SaturateOnIntegerOverflow=on  OutDataTypeStr=Inherit: Same as first input
  Sum4 : Sum  InputSameDT=on  SaturateOnIntegerOverflow=on  OutDataTypeStr=Inherit: Same as first input
  Cl : Outport
  wires:
  q_rad_s/1 -> [q_rad_s]
  vt_m_s/1 -> [vt_m_s]
  p_rad_s/1 -> [p_rad_s]
  Ail_L_deg/1 -> [Ail_L_deg]
  Ail_R_deg/1 -> [Ail_R_deg]
  MAB/1 -> [MAB]
  r_rad_s/1 -> [r_rad_s]
  Rud_deg/1 -> [Rud_deg]
  Ele_deg/1 -> [Ele_deg]
  Sum4/1 -> Cl/1
  Clq/1 -> Product2/1
  [r_rad_s] -> Product3/2
  Cld01/1 -> Product4/1
  [q_rad_s] -> Product2/2
  [Rud_deg] -> Product6/2
  [Ele_deg] -> Product5/2
  [Ail_R_deg] -> Product4/2
  [p_rad_s] -> Product1/2
  Product2/1 -> Multiply2/1
  Cld02/1 -> Product7/1
  Multiply1/1 -> Sum1/3
  [MAB] -> Clr/1, Clq/1, Clp/1, Cltot/1, Cld04/1, Cld03/1, Cld02/1, Cld01/1
  Cld04/1 -> Product6/1
  Product5/1 -> Sum of Controls/3
  [vt_m_s] -> Product10/2
  Cld03/1 -> Product5/1
  [Ail_L_deg] -> Product7/2
  Multiply/1 -> Sum1/1
  Product3/1 -> Multiply1/1
  Sum of Controls/1 -> Gain/1
  Product10/1 -> Sum of Datum/2
  Multiply2/1 -> Sum1/2
  Cltot/1 -> Sum of Datum/1
  Clr/1 -> Product3/1
  Sum1/1 -> Product10/1
  Product1/1 -> Multiply/1
  Clp/1 -> Product1/1
  Product6/1 -> Sum of Controls/4
  Sum of Datum/1 -> Sum4/1
  Gain/1 -> Sum4/2
  Product4/1 -> Sum of Controls/1
  Product7/1 -> Sum of Controls/2

== system FW_SkySurfer_HIL/UAV/UAV/Aerodynamic/Cm ==
  MAB : Inport
  vt_m_s : Inport  Port=2
  p_rad_s : Inport  Port=3
  q_rad_s : Inport  Port=4
  r_rad_s : Inport  Port=5
  Ail_R_deg : Inport  Port=6
  Ail_L_deg : Inport  Port=7
  Ele_deg : Inport  Port=8
  Rud_deg : Inport  Port=9
  Cmd01 : Lookup_n-D  NumberOfTableDimensions=3  BreakpointsForDimension1=mach_avl  BreakpointsForDimension2=alpha_avl  BreakpointsForDimension3=beta_avl  UseOneInputPortForAllInputData=on  Table=Cmd01  InternalRulePriority=Speed  RndMeth=Simplest
  Cmd02 : Lookup_n-D  NumberOfTableDimensions=3  BreakpointsForDimension1=mach_avl  BreakpointsForDimension2=alpha_avl  BreakpointsForDimension3=beta_avl  UseOneInputPortForAllInputData=on  Table=Cmd02  InternalRulePriority=Speed  RndMeth=Simplest
  Cmd03 : Lookup_n-D  NumberOfTableDimensions=3  BreakpointsForDimension1=mach_avl  BreakpointsForDimension2=alpha_avl  BreakpointsForDimension3=beta_avl  UseOneInputPortForAllInputData=on  Table=Cmd03  InternalRulePriority=Speed  RndMeth=Simplest
  Cmd04 : Lookup_n-D  NumberOfTableDimensions=3  BreakpointsForDimension1=mach_avl  BreakpointsForDimension2=alpha_avl  BreakpointsForDimension3=beta_avl  UseOneInputPortForAllInputData=on  Table=Cmd04  InternalRulePriority=Speed  RndMeth=Simplest
  Cmp : Lookup_n-D  NumberOfTableDimensions=3  BreakpointsForDimension1=mach_avl  BreakpointsForDimension2=alpha_avl  BreakpointsForDimension3=beta_avl  UseOneInputPortForAllInputData=on  Table=Cmp  InternalRulePriority=Speed  RndMeth=Simplest
  Cmq : Lookup_n-D  NumberOfTableDimensions=3  BreakpointsForDimension1=mach_avl  BreakpointsForDimension2=alpha_avl  BreakpointsForDimension3=beta_avl  UseOneInputPortForAllInputData=on  Table=Cmq  InternalRulePriority=Speed  RndMeth=Simplest
  Cmr : Lookup_n-D  NumberOfTableDimensions=3  BreakpointsForDimension1=mach_avl  BreakpointsForDimension2=alpha_avl  BreakpointsForDimension3=beta_avl  UseOneInputPortForAllInputData=on  Table=Cmr  InternalRulePriority=Speed  RndMeth=Simplest
  Cmtot : Lookup_n-D  NumberOfTableDimensions=3  BreakpointsForDimension1=mach_avl  BreakpointsForDimension2=alpha_avl  BreakpointsForDimension3=beta_avl  UseOneInputPortForAllInputData=on  Table=Cmtot  InternalRulePriority=Speed  RndMeth=Simplest
  Multiply : Gain  Gain=b/2
  Multiply1 : Gain  Gain=b/2
  Multiply2 : Gain  Gain=cbar/2
  Product{1..7} (7 alike) : Product
  Product10 : Product  Inputs=*/  InputSameDT=on  SaturateOnIntegerOverflow=on  OutDataTypeStr=Inherit: Same as first input
  Sum of Controls : Sum  Inputs=++++
  Sum of Datum : Sum
  Sum1 : Sum  Inputs=+++  InputSameDT=on  SaturateOnIntegerOverflow=on  OutDataTypeStr=Inherit: Same as first input
  Sum4 : Sum  InputSameDT=on  SaturateOnIntegerOverflow=on  OutDataTypeStr=Inherit: Same as first input
  Cm : Outport
  wires:
  q_rad_s/1 -> [q_rad_s]
  vt_m_s/1 -> [vt_m_s]
  p_rad_s/1 -> [p_rad_s]
  Ail_L_deg/1 -> [Ail_L_deg]
  Ail_R_deg/1 -> [Ail_R_deg]
  MAB/1 -> [MAB]
  r_rad_s/1 -> [r_rad_s]
  Rud_deg/1 -> [Rud_deg]
  Ele_deg/1 -> [Ele_deg]
  Product1/1 -> Multiply/1
  Cmtot/1 -> Sum of Datum/1
  Cmd04/1 -> Product6/1
  Product4/1 -> Sum of Controls/1
  Product6/1 -> Sum of Controls/4
  Multiply/1 -> Sum1/1
  Cmr/1 -> Product3/1
  [Rud_deg] -> Product6/2
  Sum of Datum/1 -> Sum4/1
  Cmp/1 -> Product1/1
  Product7/1 -> Sum of Controls/2
  Sum1/1 -> Product10/1
  Product10/1 -> Sum of Datum/2
  Sum of Controls/1 -> Sum4/2
  Cmd03/1 -> Product5/1
  [Ail_L_deg] -> Product7/2
  Multiply2/1 -> Sum1/2
  Product5/1 -> Sum of Controls/3
  Sum4/1 -> Cm/1
  Cmd02/1 -> Product7/1
  Multiply1/1 -> Sum1/3
  [MAB] -> Cmr/1, Cmq/1, Cmp/1, Cmtot/1, Cmd01/1, Cmd02/1, Cmd04/1, Cmd03/1
  Cmd01/1 -> Product4/1
  Product2/1 -> Multiply2/1
  [Ele_deg] -> Product5/2
  Cmq/1 -> Product2/1
  [Ail_R_deg] -> Product4/2
  Product3/1 -> Multiply1/1
  [r_rad_s] -> Product3/2
  [p_rad_s] -> Product1/2
  [q_rad_s] -> Product2/2
  [vt_m_s] -> Product10/2
